simulink model "simulator_model_controller_compliance1"  (R2023b)
settings: Solver=ode4  StartTime=0.0  StopTime=5  FixedStep=0.001  MaxStep=0.01  RelTol=1e-3
values from neighbouring files (symbols this model uses):
  Fc = Simulink.Parameter([0; 0])    [main.m]
  Fv = 0.04    [main.m]
  g = Simulink.Parameter(9.81)    [main.m]
  I1 = Simulink.Parameter( (1/12)*m1.Value*(l1.Value^2) )    [main.m]
  I2 = Simulink.Parameter( (1/12)*m2.Value*(l2.Value^2) )    [main.m]
  Kd = sqrt(Kp/3)*3    [main.m]
  ke = Simulink.Parameter([Ks 0 ; 0 Ks])    [main.m]
  Kp = 10    [main.m]
  l1 = Simulink.Parameter(1)    [main.m]    (also in plot_robot.m = inputs(3); plot_robot_3links.m = inputs(4))
  l2 = Simulink.Parameter(1)    [main.m]    (also in plot_robot.m = inputs(4); plot_robot_3links.m = inputs(5))
  lc1 = Simulink.Parameter(l1.Value/2)    [main.m]
  lc2 = Simulink.Parameter(l2.Value/2)    [main.m]
  m1 = Simulink.Parameter(0.5)    [main.m]
  m2 = Simulink.Parameter(0.2)    [main.m]
  Xe = Simulink.Parameter([0.2 ; -0.2])    [main.m]
settings Model: Creator=Gabriel  LastModifiedBy=Bruno
settings DebuggingCC: SignalInfNanChecking=error

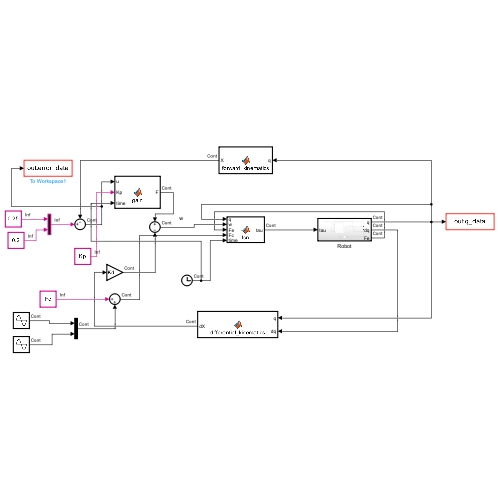
[thumbnail: Simulink's stored preview of the top-level diagram]
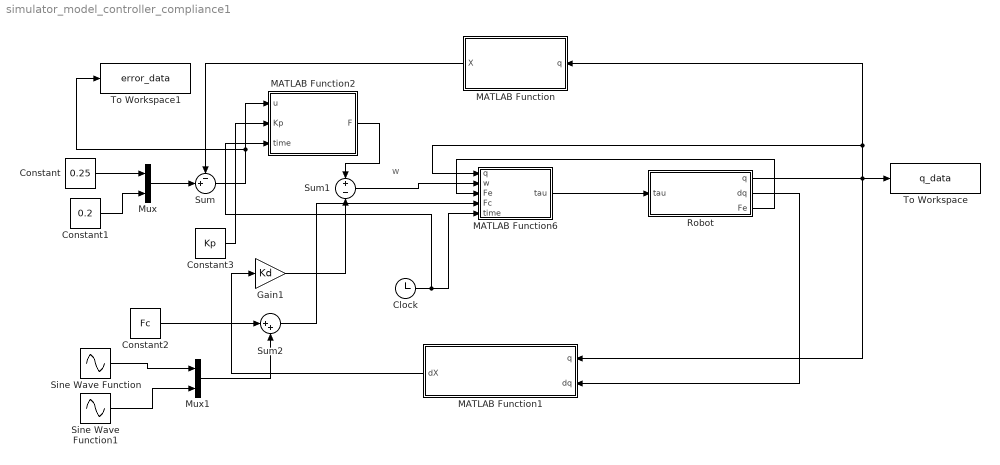
== system simulator_model_controller_compliance1 ==
  note: w
  Clock : Clock
  Constant : Constant  Value=0.25
  Constant1 : Constant  Value=0.2
  Constant2 : Constant  Value=Fc
  Constant3 : Constant  Value=Kp
  Gain1 : Gain  Gain=Kd
  MATLAB Function : MATLAB Function  TreatAsAtomicUnit=on
  MATLAB Function1 : MATLAB Function  TreatAsAtomicUnit=on
  MATLAB Function2 : MATLAB Function  TreatAsAtomicUnit=on
  MATLAB Function6 : MATLAB Function  TreatAsAtomicUnit=on
  Mux : Mux  Inputs=2
  Mux1 : Mux  Inputs=2
  Robot : Subsystem
  Sine Wave Function : Sin  Amplitude=0  SampleTime=0
  Sine Wave Function1 : Sin  Amplitude=20  Frequency=2*pi  SampleTime=0
  Sum : Sum  Inputs=-+|
  Sum1 : Sum  Inputs=+-
  Sum2 : Sum  Inputs=|++
  To Workspace : ToWorkspace  VariableName=q_data  SampleTime=-1
      settings: Save2DSignal=2-D array (concatenate along first dimension)
  To Workspace1 : ToWorkspace  VariableName=error_data  SampleTime=-1
      settings: Save2DSignal=2-D array (concatenate along first dimension)
  wires:
  MATLAB Function/1(X) -> Sum/1
  Gain1/1 -> Sum1/2
  Sum/1 -> To Workspace1/1, MATLAB Function2/1(u)
  Robot/2(dq) -> MATLAB Function1/2(dq)
  MATLAB Function1/1(dX) -> Gain1/1
  Sum1/1 -> MATLAB Function6/2(w)
  Robot/3(Fe) -> MATLAB Function6/3(Fe)
  MATLAB Function6/1(tau) -> Robot/1(tau)
  Mux/1 -> Sum/2
  Robot/1(q) -> MATLAB Function6/1(q), MATLAB Function/1(q), To Workspace/1, MATLAB Function1/1(q)
  Constant/1 -> Mux/1
  Constant1/1 -> Mux/2
  Constant2/1 -> Sum2/1
  Sine Wave Function/1 -> Mux1/1
  Sine Wave Function1/1 -> Mux1/2
  Mux1/1 -> Sum2/2
  Sum2/1 -> MATLAB Function6/4(Fc)
  MATLAB Function2/1(F) -> Sum1/1
  Constant3/1 -> MATLAB Function2/2(Kp)
  Clock/1 -> MATLAB Function2/3(time), MATLAB Function6/5(time)

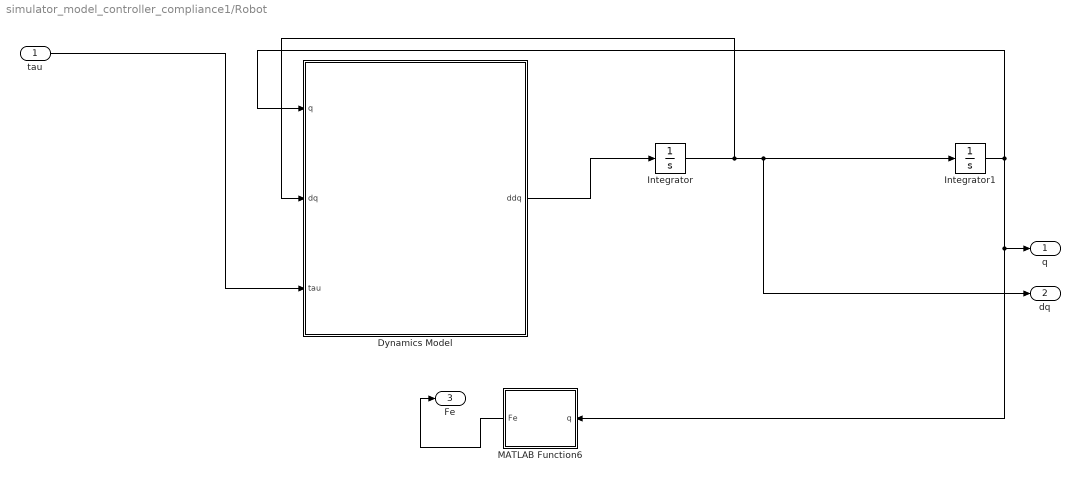
== system simulator_model_controller_compliance1/Robot ==
  tau : Inport
  Dynamics Model : MATLAB Function  TreatAsAtomicUnit=on
  Integrator : Integrator  InitialCondition=[0;0]
  Integrator1 : Integrator  InitialCondition=[pi/2;pi/4]
  MATLAB Function6 : MATLAB Function  TreatAsAtomicUnit=on
  q : Outport
  dq : Outport  Port=2
  Fe : Outport  Port=3
  wires:
  Integrator1/1 -> MATLAB Function6/1(q), q/1, Dynamics Model/1(q)
  tau/1 -> Dynamics Model/3(tau)
  Dynamics Model/1(ddq) -> Integrator/1
  Integrator/1 -> Dynamics Model/2(dq), dq/1, Integrator1/1
  MATLAB Function6/1(Fe) -> Fe/1

== matlab function simulator_model_controller_compliance1/Robot/Dynamics Model ==
  data: q input; ddq output; dq input; tau input; m1 parameter; m2 parameter; l1 parameter; l2 parameter; lc1 parameter; lc2 parameter; I1 parameter; I2 parameter; g parameter; Fv parameter
function ddq = dynamics(q,dq,tau,m1, m2, l1, l2, lc1, lc2, I1, I2, g, Fv)

    M = mass_matrix(q(1),q(2),m1,m2,l1,l2,lc1,lc2,I1,I2);
    C = coriolis_matrix(q(1),q(2),dq(1),dq(2),m1,m2,l1,l2,lc1,lc2);
    G = gravity_vector(q(1),q(2),m1,m2,l1,l2,lc1,lc2,g);
    
    %--------------------------------------------
    %     REGULARIZAÇÃO PARA EVITAR SINGULARIDADES
    %--------------------------------------------
    cond_min = 1e-6;       % limite antes de considerar a matriz perigosa
    eps_reg  = 1e-6;       % força de regularização

    if rcond(M) < cond_min
        M = M + eps_reg * eye(2);
    end

    %--------------------------------------------
    %     CÁLCULO DAS ACELERAÇÕES
    %--------------------------------------------
    ddq = M \ (tau - C*dq - G - Fv*dq);

    %--------------------------------------------
    %     LIMITAÇÃO PARA EVITAR EXPLOSÕES NUMÉRICAS
    %--------------------------------------------
    ddq_max = 1e4;
    ddq = min(max(ddq, -ddq_max), ddq_max);

end

== matlab function simulator_model_controller_compliance1/MATLAB Function ==
  data: q input; l1 parameter; X output; l2 parameter
function X  = forward_kinematics(q, l1,l2)
    X=forward_kinematics(q(1),q(2),l1,l2);

== matlab function simulator_model_controller_compliance1/MATLAB Function1 ==
  data: q input; dX output; dq input; l1 parameter; l2 parameter
function dX  = differential_kinematics(q,dq, l1, l2)
            q1=q(1);
            q2=q(2);
            J=Jacobian.linear_jacobian(q1,q2,l1,l2);
            dX = J*dq;

== matlab function simulator_model_controller_compliance1/MATLAB Function2 ==
  data: u input; F output; Kp input; kp parameter; time input
function F = gain(u,Kp, kp, time)

if time<1
    F=Kp*u;
else 
    F=kp*u;
end

== matlab function simulator_model_controller_compliance1/MATLAB Function6 ==
  data: q input; tau output; w input; Fe input; m2 parameter; l1 parameter; l2 parameter; lc1 parameter; lc2 parameter; g parameter; m1 parameter; Fc input; Xe parameter; time input
function tau = fcn(q,w,Fe, m2, l1, l2, lc1, lc2, g, m1, Fc, Xe, time)
G = gravity_vector(q(1),q(2),m1,m2,l1,l2,lc1,lc2,g);
J=Jacobian.linear_jacobian(q(1),q(2),l1,l2);
X=forward_kinematics(q(1),q(2),l1,l2);

F_bone=J'*Fe;
y=J'*w;
if time >= 1
    F_surgeon = Fc;
else 
    F_surgeon = [0;0];

end


tau=y+G+J'*F_surgeon-F_bone;

== matlab function simulator_model_controller_compliance1/Robot/MATLAB Function6 ==
  data: q input; Fe output; l1 parameter; l2 parameter; Xe parameter; ke parameter
function Fe = force_environment(q, l1, l2, Xe, ke)
    % Posição do end-effector
    X = forward_kinematics(q(1), q(2), l1, l2);
    if (X(1) - Xe(1)) >= 0
    % Contacto (penetração no osso)
        Fe_compliance = [ke(1,1) * (X(1) - Xe(1)); 0];
    else
    
        Fe_compliance = [0; 0];
    end
    
    % Soma de todas as forças
    Fe = Fe_compliance;
end
